simulink model "DCMotor_Lab4_Soln"  (R2023b)
settings: Solver=VariableStepAuto  StartTime=0.0  StopTime=5  MaxStep=0.001  RelTol=1e-3
PostLoadFcn:
  | % Resize the model window
  | set(0,"Units","pixels")
  | sSize = get(0,"screensize");
  | set_param(gcs,'location',...
  |     [1,sSize(4)*0.01,round(sSize(3)/2),sSize(4)*0.96]);
values from neighbouring files (symbols this model uses):
  m = 1000    [VehicleModelSoln.m]
  s = tf('s')    [PositionAnalysisSoln.m]
undefined symbols (not defined in the file or in its folder): X, Y, Z
libraries: sm_lib x22, fl_lib x10, nesl_utility x3, simulink_extras x1, simulink x1
settings Model: Creator=Rocksmithed  LastModifiedBy=callie
settings DebuggingCC: UnconnectedInputMsg=warning  UnconnectedOutputMsg=warning  UnconnectedLineMsg=warning
settings ModelReferenceCC: EnableRefExpFcnMdlSchedulingChecks=on
settings RTWCC: DLArmComputeVersion=19.05
settings ExplorerConfigSet: InternalSimMechanicsExplorerSettings="<ExplorerConfiguration><canonicalview>default</canonicalview><AnimationSetting><BasePlaybackSpeed>1.0</BasePlaybackSpeed><PlaybackSpeedFactor>1.0</PlaybackSpeedFactor></AnimationSetting><TilePanel><TileInfo><Tiles Columns=\"1\" Count=\"2\" Rows=\"2\"><Column Weight=\"1\"/><Row Weight=\"0.567\"/><Row Weight=\"0.433\"/><Tile Height=\"1\" Width=\"1\" X=\"0\" Y=\"0\"/><Tile Height=\"1\" Width=\"1\" X=\"0\" Y=\"1\"/></Tiles></TileInfo><SceneInfo><SceneViewer><BGColor><R>0.941176474094390869</R><G>0.941176474094390869</G><B>0.941176474094390869</B></BGColor><Camera><DoPerspective>off</DoPerspective><Position><X>-0.000930544299837629606</X><Y>-0.991947113333839781</Y><Z>-0.000895731694159566396</Z></Position><Center><X>-0.000930544299837629606</X><Y>0.00805288666616021942</Y><Z>-0.000895731694159566396</Z></Center><Up><X>0</X><Y>-0</Y><Z>1</Z></Up><ViewLimDist>1</ViewLimDist><YLim>0.032783521950277443</YLim><XLim>0.0566081835477763654</XLim></Camera></SceneViewer><SceneViewer><BGColor><R>0.941176474094390869</R><G>0.941176474094390869</G><B>0.941176474094390869</B></BGColor><Camera><DoPerspective>off</DoPerspective><Position><X>0.999997946466442578</X><Y>0.00754476683050594576</Y><Z>-0.00157074132845253563</Z></Position><Center><X>-2.05353355742232679e-06</X><Y>0.00754476683050594576</Y><Z>-0.00157074132845253563</Z></Center><Up><X>-0</X><Y>0</Y><Z>1</Z></Up><ViewLimDist>1</ViewLimDist><YLim>0.029549906028231071</YLim><XLim>0.0669823756881716137</XLim></Camera></SceneViewer></SceneInfo></TilePanel><MechEditorPanel><Cameras/><GfxPanelCameraMap/><VideoCreator><PlaybackSpeedRatio>1.0</PlaybackSpeedRatio><FrameRate>30</FrameRate><VideoFormat>Motion JPEG AVI</VideoFormat><FrameSize>auto</FrameSize></VideoCreator></MechEditorPanel></ExplorerConfiguration>"

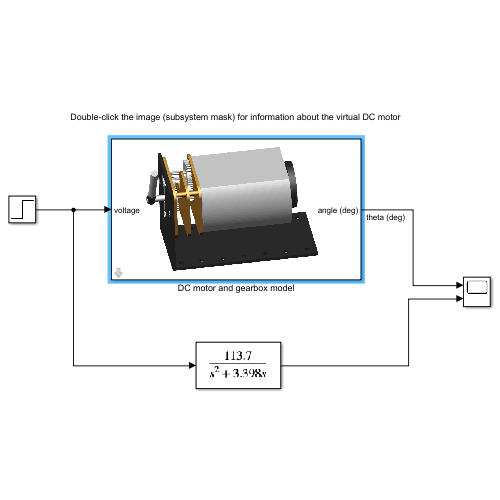
[thumbnail: Simulink's stored preview of the top-level diagram]
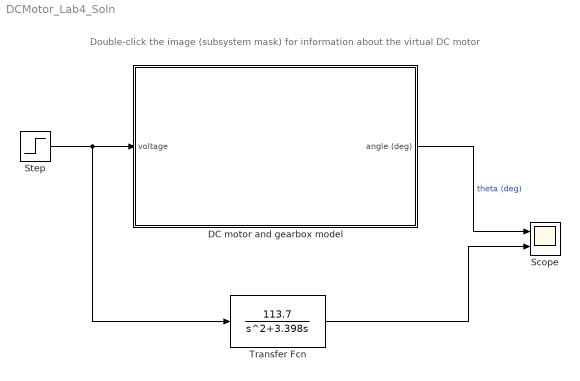
== system DCMotor_Lab4_Soln ==
  note: Double-click the image (subsystem mask) for information about the virtual DC motor
  DC motor and gearbox model : Subsystem  mask{B=0.028, K=0.05, L=0.1, R=0.25, noiseGain=0, saturationOn=off, pmass=0.150, plength=0.015}
      mask prompts: B "B: damping (N*m/(rad/s))"; K "K: constant of proportionality [V/(rad/s)]"; L "L: inductance (H)"; R "R: resistance (ohm)"; noiseGain "Sensor noise gain"; saturationOn "Use voltage saturation"; pmass "Pendulum mass (kg)"; plength "Pendulum length (m)"
      mask help:
      | This block implements a virtual DC motor using Simscape Multibody. The motor has a speed reducer with a 9:1 gear ratio.
      |
      | Inputs:
      |   voltage: the voltage applied to the motor in volts.
      | Outputs:
      |   angle: the angle of the output shaft in degrees.
      mask DialogControl Motor Prompt: Motor
      mask DialogControl Pendulum Prompt: Pendulum
      mask Display: image('dcmotor.png');
  Scope : Scope  NumInputPorts=2
  Step : Step  Time=0  SampleTime=0
  Transfer Fcn : TransferFcn  Numerator=[113.7]  Denominator=[1 3.398 0]
  wires:
  Step/1 -> Transfer Fcn/1, DC motor and gearbox model/1(voltage)
  DC motor and gearbox model/1(angle (deg)) -> Scope/1  "theta (deg)"
  Transfer Fcn/1 -> Scope/2

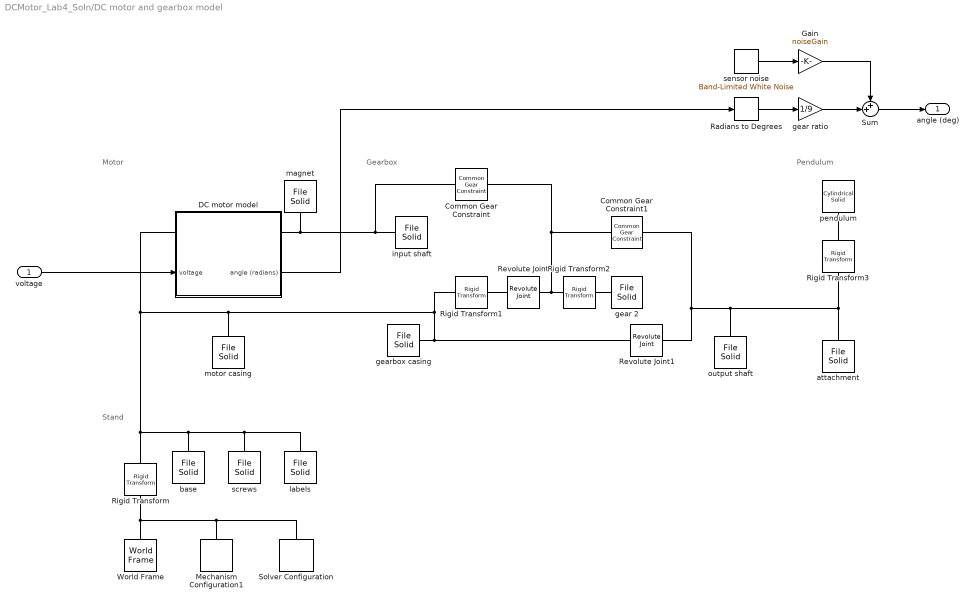
== system DCMotor_Lab4_Soln/DC motor and gearbox model ==
  note: Motor
  note: Stand
  note: Gearbox
  note: Pendulum
  voltage : Inport
  Common Gear Constraint : sm_lib/Gears and Couplings/Gears/Common Gear Constraint  GearType=External  SpecificationType=CenterDistanceRatio  CenterDistance=sqrt( 0.0046^2 + 0.0029^2 )  CenterDistanceUnits=m  GearRatio=3  BaseGearRadius=0.084  BaseGearRadiusUnits=m  FollGearRadius=0.084/3  FollGearRadiusUnits=cm  AssemblyGearRotation=Free
  Common Gear Constraint1 : sm_lib/Gears and Couplings/Gears/Common Gear Constraint  GearType=External  SpecificationType=CenterDistanceRatio  CenterDistance=sqrt( 0.0046^2 + 0.0029^2 )  CenterDistanceUnits=m  GearRatio=3  BaseGearRadius=0.084  BaseGearRadiusUnits=m  FollGearRadius=0.084/3  FollGearRadiusUnits=cm  AssemblyGearRotation=Free
  DC motor model : Subsystem
      settings: PortSchema="{\"entries\":[{\"content\":{\"sides\":[{\"content\":{\"connectorIds\":[\"LConn1\",\"In1\"]},\"type\":\"ConnectorPlacement.EquallySpacedRectSide\",\"uuid\":\"5a6d496b-9b68-4e77-90bc-41353dc42901\"},{\"content\":{\"connectorIds\":[\"RConn1\",\"Out1\"],\"side\":\"RIGHT\"},\"type\":\"ConnectorPlacement.EquallySpacedRectSide\",\"uuid\":\"9792b535-129a-41a8-a62b-92ba389600f0\"},{\"content\":{\"connectorIds\":[],\"side\":\"TOP\"},\"type\":\"ConnectorPlacement.EquallySpacedRectSide\",\"uuid\":\"2aab1536-3ac2-4e27-9370-d50050e6f4f6\"}]},\"type\":\"ConnectorPlacement.EquallySpacedConnector\",\"uuid\":\"df64eeb9-387f-493f-b882-741ae516d086\"}],\"packageUris\":[\"http://schema.mathworks.com/mf0/Connector/R2020b\"],\"version\":\"1.0\"}"
  Gain : Gain  Gain=noiseGain
  Mechanism Configuration1 : sm_lib/Utilities/Mechanism Configuration  UniformGravity=Constant  GravityVector=[0 0 -9.80665]  GravityVectorUnits=m/s^2  GravityUnits=m/s^2  LinearizationDelta=0.001  JointModeTransitionNonlinearIterations=2
  Radians to Degrees : simulink_extras/Transformations/Radians to Degrees
  Revolute Joint : sm_lib/Joints/Revolute Joint  JointMode=Normal  SenseConstraintForce=off  SenseConstraintForceX=off  SenseConstraintForceY=off  SenseConstraintForceZ=off  SenseConstraintTorque=off  SenseConstraintTorqueX=off  SenseConstraintTorqueY=off  SenseConstraintTorqueZ=off  SenseTotalForce=off  SenseTotalForceX=off  SenseTotalForceY=off  SenseTotalForceZ=off  SenseTotalTorque=off  SenseTotalTorqueX=off  SenseTotalTorqueY=off  SenseTotalTorqueZ=off  CompositeWrenchDir=FollowerOnBase  CompositeWrenchFrame=BaseFrame  EquilibriumPosition=0  EquilibriumPositionUnits=deg  SpringStiffness=0  SpringStiffnessUnits=N*m/deg  DampingCoefficient=0  DampingCoefficientUnits=N*m/(deg/s)  TorqueActuationMode=NoTorque  MotionActuationMode=ComputedMotion  SensePosition=off  SenseVelocity=off  SenseAcceleration=off  SenseTorqueForce=off  SenseLowerLimitTorqueForce=off  SenseUpperLimitTorqueForce=off  LowerLimitSpecify=off  LowerLimitBound=-90  LowerLimitBoundUnits=deg  LowerLimitStiffness=1e4  LowerLimitStiffnessUnits=N*m/deg  LowerLimitDamping=10  LowerLimitDampingUnits=N*m/(deg/s)  LowerLimitTransitionRegionWidth=0.1  LowerLimitTransitionRegionWidthUnits=deg  UpperLimitSpecify=off  UpperLimitBound=90  UpperLimitBoundUnits=deg  UpperLimitStiffness=1e4  UpperLimitStiffnessUnits=N*m/deg  UpperLimitDamping=10  UpperLimitDampingUnits=N*m/(deg/s)  UpperLimitTransitionRegionWidth=0.1  UpperLimitTransitionRegionWidthUnits=deg  PositionTargetSpecify=off  PositionTargetPriority=High  PositionTargetValue=0  PositionTargetValueUnits=deg  VelocityTargetSpecify=off  VelocityTargetPriority=High  VelocityTargetValue=0  VelocityTargetValueUnits=deg/s
  Revolute Joint1 : sm_lib/Joints/Revolute Joint  JointMode=Normal  SenseConstraintForce=off  SenseConstraintForceX=off  SenseConstraintForceY=off  SenseConstraintForceZ=off  SenseConstraintTorque=off  SenseConstraintTorqueX=off  SenseConstraintTorqueY=off  SenseConstraintTorqueZ=off  SenseTotalForce=off  SenseTotalForceX=off  SenseTotalForceY=off  SenseTotalForceZ=off  SenseTotalTorque=off  SenseTotalTorqueX=off  SenseTotalTorqueY=off  SenseTotalTorqueZ=off  CompositeWrenchDir=FollowerOnBase  CompositeWrenchFrame=BaseFrame  EquilibriumPosition=0  EquilibriumPositionUnits=deg  SpringStiffness=0  SpringStiffnessUnits=N*m/deg  DampingCoefficient=0  DampingCoefficientUnits=N*m/(deg/s)  TorqueActuationMode=NoTorque  MotionActuationMode=ComputedMotion  SensePosition=off  SenseVelocity=off  SenseAcceleration=off  SenseTorqueForce=off  SenseLowerLimitTorqueForce=off  SenseUpperLimitTorqueForce=off  LowerLimitSpecify=off  LowerLimitBound=-90  LowerLimitBoundUnits=deg  LowerLimitStiffness=1e4  LowerLimitStiffnessUnits=N*m/deg  LowerLimitDamping=10  LowerLimitDampingUnits=N*m/(deg/s)  LowerLimitTransitionRegionWidth=0.1  LowerLimitTransitionRegionWidthUnits=deg  UpperLimitSpecify=off  UpperLimitBound=90  UpperLimitBoundUnits=deg  UpperLimitStiffness=1e4  UpperLimitStiffnessUnits=N*m/deg  UpperLimitDamping=10  UpperLimitDampingUnits=N*m/(deg/s)  UpperLimitTransitionRegionWidth=0.1  UpperLimitTransitionRegionWidthUnits=deg  PositionTargetSpecify=off  PositionTargetPriority=High  PositionTargetValue=0  PositionTargetValueUnits=deg  VelocityTargetSpecify=off  VelocityTargetPriority=High  VelocityTargetValue=0  VelocityTargetValueUnits=deg/s
  Rigid Transform : sm_lib/Frames and Transforms/Rigid Transform  TranslationMethod=None  TranslationStandardOffset=0  TranslationLengthUnit=m  TranslationStandardAxis=+Z  TranslationCartesianOffset=[0 0 0]  TranslationROffset=0  TranslationROffsetUnits=m  TranslationZOffset=0  TranslationZOffsetUnits=m  TranslationThetaOffset=0  TranslationThetaOffsetUnits=deg  RotationMethod=StandardAxis  RotationAngleUnits=deg  RotationStandardAxis=+X  RotationAngle=90  RotationArbitraryAxis=[0 0 1]  FollAlignAxisA=+X  BaseAlignAxisA=+Y  FollAlignAxisB=+Y  BaseAlignAxisB=+Z  RotationSequenceAxes=FollowerAxes  RotationSequence=XYX  RotationSequenceAngles=[0 0 0]  RotationSequenceAnglesUnits=deg  RotationMatrix=[1 0 0; 0 1 0; 0 0 1]
  Rigid Transform1 : sm_lib/Frames and Transforms/Rigid Transform  TranslationMethod=Cartesian  TranslationStandardOffset=0  TranslationLengthUnit=m  TranslationStandardAxis=+Z  TranslationCartesianOffset=[-0.0046 0.0029 0]  TranslationROffset=0  TranslationROffsetUnits=m  TranslationZOffset=0  TranslationZOffsetUnits=m  TranslationThetaOffset=0  TranslationThetaOffsetUnits=deg  RotationMethod=None  RotationAngleUnits=deg  RotationStandardAxis=+Z  RotationAngle=0.0  RotationArbitraryAxis=[0 0 1]  FollAlignAxisA=+X  BaseAlignAxisA=+Y  FollAlignAxisB=+Y  BaseAlignAxisB=+Z  RotationSequenceAxes=FollowerAxes  RotationSequence=XYX  RotationSequenceAngles=[0 0 0]  RotationSequenceAnglesUnits=deg  RotationMatrix=[1 0 0; 0 1 0; 0 0 1]
  Rigid Transform2 : sm_lib/Frames and Transforms/Rigid Transform  TranslationMethod=Cartesian  TranslationStandardOffset=0  TranslationLengthUnit=m  TranslationStandardAxis=+Z  TranslationCartesianOffset=[-0.0046 0.0029 0]  TranslationROffset=0  TranslationROffsetUnits=m  TranslationZOffset=0  TranslationZOffsetUnits=m  TranslationThetaOffset=0  TranslationThetaOffsetUnits=deg  RotationMethod=None  RotationAngleUnits=deg  RotationStandardAxis=+Z  RotationAngle=0.0  RotationArbitraryAxis=[0 0 1]  FollAlignAxisA=+X  BaseAlignAxisA=+Y  FollAlignAxisB=+Y  BaseAlignAxisB=+Z  RotationSequenceAxes=FollowerAxes  RotationSequence=XYX  RotationSequenceAngles=[0 0 0]  RotationSequenceAnglesUnits=deg  RotationMatrix=[1 0 0; 0 1 0; 0 0 1]
  Rigid Transform3 : sm_lib/Frames and Transforms/Rigid Transform  TranslationMethod=Cartesian  TranslationStandardOffset=0  TranslationLengthUnit=m  TranslationStandardAxis=+Z  TranslationCartesianOffset=[0, -plength/2, 0.01075]  TranslationROffset=0  TranslationROffsetUnits=m  TranslationZOffset=0  TranslationZOffsetUnits=m  TranslationThetaOffset=0  TranslationThetaOffsetUnits=deg  RotationMethod=StandardAxis  RotationAngleUnits=deg  RotationStandardAxis=+X  RotationAngle=90  RotationArbitraryAxis=[0 0 1]  FollAlignAxisA=+X  BaseAlignAxisA=+Y  FollAlignAxisB=+Y  BaseAlignAxisB=+Z  RotationSequenceAxes=FollowerAxes  RotationSequence=XYX  RotationSequenceAngles=[0 0 0]  RotationSequenceAnglesUnits=deg  RotationMatrix=[1 0 0; 0 1 0; 0 0 1]
  Solver Configuration : nesl_utility/Solver Configuration  PhysicalDomain=network_engine_domain  SubClassName=solver  LeftPortType=input  RightPortType=generic  Tones=[]  Harmonics=[]  SimulateNoise=off  Profile=off  UseLocalSampling=off  EnableSwitchedLinearOptims=on  FrequencyDomain=off  UseCCode=off  RelTol=0.001  AbsTol=1e-06  MinStep=1e-09  ToWorkspace=off  RevertToSquareIcSolve=off  NumHomotopyIterations=100  PhasorMode=off  PhasorModeNumHarmonics=1  DoDC=off  ResidualTolerance=1e-09  UseLocalSolver=off  LocalSolverChoice=NE_BACKWARD_EULER_ADVANCER  LocalSolverSampleTime=0.001  DoFixedCost=off  MaxNonlinIter=3  MaxModeIter=2  ComputeImpulses=off  ImpulseIterations=2  LinearAlgebra=Sparse  EquationFormulation=NE_TIME_EF  DelaysMemoryBudget=1024  AutomaticFiltering=on  FilteringTimeConstant=0.001  PartitionStorageMethod=AS_NEEDED  PartitionMemoryBudget=1024  PartitionMethod=FAST
  Sum : Sum  Inputs=++|
  World Frame : sm_lib/Frames and Transforms/World Frame
  attachment : sm_lib/Body Elements/File Solid  ExtGeomFileName=dc_pendulumattachment.stl  UnitType=Custom  ExtGeomFileUnits=m  StepReaderType=HEX  ExportConvexHullGeometry=off  InertiaType=CalculateFromGeometry  Mass=1  MassUnits=kg  CenterOfMass=[0 0 0]  CenterOfMassUnits=m  MomentsOfInertia=[1 1 1]  MomentsOfInertiaUnits=kg*m^2  ProductsOfInertia=[0 0 0]  ProductsOfInertiaUnits=kg*m^2  BasedOnType=Density  Density=1000  DensityUnits=kg/m^3  DoExposeReferenceFrame=on  SerializedFrames=<Frames/>  GraphicType=FromGeometry  MarkerShape=Sphere  MarkerSize=10  GraphicVisPropType=AdvancedVisualProperties  GraphicDiffuseColor=[0.1 0.1 0.1 1]  GraphicSpecularColor=[0.9 0.9 0.9 1]  GraphicAmbientColor=[0.1 0.1 0.1 1]  GraphicEmissiveColor=[0 0 0 1]  GraphicShininess=10  GraphicOpacity=1.0
  base : sm_lib/Body Elements/File Solid  ExtGeomFileName=dc_stand.stl  UnitType=Custom  ExtGeomFileUnits=m  StepReaderType=HEX  ExportConvexHullGeometry=off  InertiaType=CalculateFromGeometry  Mass=1  MassUnits=kg  CenterOfMass=[0 0 0]  CenterOfMassUnits=m  MomentsOfInertia=[1 1 1]  MomentsOfInertiaUnits=kg*m^2  ProductsOfInertia=[0 0 0]  ProductsOfInertiaUnits=kg*m^2  BasedOnType=Density  Density=1000  DensityUnits=kg/m^3  DoExposeReferenceFrame=on  SerializedFrames=<Frames/>  GraphicType=FromGeometry  MarkerShape=Sphere  MarkerSize=10  GraphicVisPropType=AdvancedVisualProperties  GraphicDiffuseColor=[0.1 0.1 0.1 1]  GraphicSpecularColor=[0.9 0.9 0.9 1]  GraphicAmbientColor=[0.1 0.1 0.1 1]  GraphicEmissiveColor=[0 0 0 1]  GraphicShininess=10  GraphicOpacity=1.0
  gear 2 : sm_lib/Body Elements/File Solid  ExtGeomFileName=dc_gear2.stl  UnitType=Custom  ExtGeomFileUnits=m  StepReaderType=HEX  ExportConvexHullGeometry=off  InertiaType=CalculateFromGeometry  Mass=1  MassUnits=kg  CenterOfMass=[0 0 0]  CenterOfMassUnits=m  MomentsOfInertia=[1 1 1]  MomentsOfInertiaUnits=kg*m^2  ProductsOfInertia=[0 0 0]  ProductsOfInertiaUnits=kg*m^2  BasedOnType=Density  Density=1000  DensityUnits=kg/m^3  DoExposeReferenceFrame=on  SerializedFrames=<Frames/>  GraphicType=FromGeometry  MarkerShape=Sphere  MarkerSize=10  GraphicVisPropType=AdvancedVisualProperties  GraphicDiffuseColor=[1,1,1]  GraphicSpecularColor=[0.7 0.7 0.7]  GraphicAmbientColor=[0.2 0.2 0.2,1]  GraphicEmissiveColor=[0,0,0,1]  GraphicShininess=5  GraphicOpacity=1.0
  gear ratio : Gain  Gain=1/9
  gearbox casing : sm_lib/Body Elements/File Solid  ExtGeomFileName=dc_gearbox.stl  UnitType=Custom  ExtGeomFileUnits=m  StepReaderType=HEX  ExportConvexHullGeometry=off  InertiaType=CalculateFromGeometry  Mass=1  MassUnits=kg  CenterOfMass=[0 0 0]  CenterOfMassUnits=m  MomentsOfInertia=[1 1 1]  MomentsOfInertiaUnits=kg*m^2  ProductsOfInertia=[0 0 0]  ProductsOfInertiaUnits=kg*m^2  BasedOnType=Density  Density=1000  DensityUnits=kg/m^3  DoExposeReferenceFrame=on  SerializedFrames=<Frames/>  GraphicType=FromGeometry  MarkerShape=Sphere  MarkerSize=10  GraphicVisPropType=AdvancedVisualProperties  GraphicDiffuseColor=[1,0.85,0.2]  GraphicSpecularColor="[1    0.9   0.8 1]"  GraphicAmbientColor=[0.15 0.05 0.05 1]  GraphicEmissiveColor=[0.0 0.0 0.0 1.0]  GraphicShininess=5  GraphicOpacity=1.0
  input shaft : sm_lib/Body Elements/File Solid  ExtGeomFileName=dc_gear1.stl  UnitType=Custom  ExtGeomFileUnits=m  StepReaderType=HEX  ExportConvexHullGeometry=off  InertiaType=CalculateFromGeometry  Mass=1  MassUnits=kg  CenterOfMass=[0 0 0]  CenterOfMassUnits=m  MomentsOfInertia=[1 1 1]  MomentsOfInertiaUnits=kg*m^2  ProductsOfInertia=[0 0 0]  ProductsOfInertiaUnits=kg*m^2  BasedOnType=Density  Density=1000  DensityUnits=kg/m^3  DoExposeReferenceFrame=on  SerializedFrames=<Frames/>  GraphicType=FromGeometry  MarkerShape=Sphere  MarkerSize=10  GraphicVisPropType=AdvancedVisualProperties  GraphicDiffuseColor=[1,1,1]  GraphicSpecularColor=[0.7 0.7 0.7]  GraphicAmbientColor=[0.2 0.2 0.2,1]  GraphicEmissiveColor=[0,0,0,1]  GraphicShininess=5  GraphicOpacity=1.0
  labels : sm_lib/Body Elements/File Solid  ExtGeomFileName=dc_labels.stl  UnitType=Custom  ExtGeomFileUnits=m  StepReaderType=HEX  ExportConvexHullGeometry=off  InertiaType=CalculateFromGeometry  Mass=1  MassUnits=kg  CenterOfMass=[0 0 0]  CenterOfMassUnits=m  MomentsOfInertia=[1 1 1]  MomentsOfInertiaUnits=kg*m^2  ProductsOfInertia=[0 0 0]  ProductsOfInertiaUnits=kg*m^2  BasedOnType=Density  Density=1000  DensityUnits=kg/m^3  DoExposeReferenceFrame=on  SerializedFrames=<Frames/>  GraphicType=FromGeometry  MarkerShape=Sphere  MarkerSize=10  GraphicVisPropType=AdvancedVisualProperties  GraphicDiffuseColor=[0.95,0.95,0.95]  GraphicSpecularColor="[0.9    0.9  0.9 1]"  GraphicAmbientColor=[0.07 0.07 0.07]  GraphicEmissiveColor=[0.0 0.0 0.0 1.0]  GraphicShininess=2  GraphicOpacity=1.0
  magnet : sm_lib/Body Elements/File Solid  ExtGeomFileName=dc_magnet.stl  UnitType=Custom  ExtGeomFileUnits=m  StepReaderType=HEX  ExportConvexHullGeometry=off  InertiaType=CalculateFromGeometry  Mass=1  MassUnits=kg  CenterOfMass=[0 0 0]  CenterOfMassUnits=m  MomentsOfInertia=[1 1 1]  MomentsOfInertiaUnits=kg*m^2  ProductsOfInertia=[0 0 0]  ProductsOfInertiaUnits=kg*m^2  BasedOnType=Density  Density=1000  DensityUnits=kg/m^3  DoExposeReferenceFrame=on  SerializedFrames=<Frames/>  GraphicType=FromGeometry  MarkerShape=Sphere  MarkerSize=10  GraphicVisPropType=AdvancedVisualProperties  GraphicDiffuseColor=[0.1 0.1 0.1 1]  GraphicSpecularColor=[0.9 0.9 0.9 1]  GraphicAmbientColor=[0.1 0.1 0.1 1]  GraphicEmissiveColor=[0 0 0 1]  GraphicShininess=10  GraphicOpacity=1.0
  motor casing : sm_lib/Body Elements/File Solid  ExtGeomFileName=dc_motorcasing.stl  UnitType=Custom  ExtGeomFileUnits=m  StepReaderType=HEX  ExportConvexHullGeometry=off  InertiaType=CalculateFromGeometry  Mass=1  MassUnits=kg  CenterOfMass=[0 0 0]  CenterOfMassUnits=m  MomentsOfInertia=[1 1 1]  MomentsOfInertiaUnits=kg*m^2  ProductsOfInertia=[0 0 0]  ProductsOfInertiaUnits=kg*m^2  BasedOnType=Density  Density=1000  DensityUnits=kg/m^3  DoExposeReferenceFrame=on  SerializedFrames=<Frames/>  GraphicType=FromGeometry  MarkerShape=Sphere  MarkerSize=10  GraphicVisPropType=AdvancedVisualProperties  GraphicDiffuseColor=[1,1,1]  GraphicSpecularColor=[0.9 0.9 0.9]  GraphicAmbientColor=[0.3 0.3 0.3]  GraphicEmissiveColor=[0,0,0,1]  GraphicShininess=25  GraphicOpacity=1.0
  output shaft : sm_lib/Body Elements/File Solid  ExtGeomFileName=dc_outputshaft.stl  UnitType=Custom  ExtGeomFileUnits=m  StepReaderType=HEX  ExportConvexHullGeometry=off  InertiaType=CalculateFromGeometry  Mass=1  MassUnits=kg  CenterOfMass=[0 0 0]  CenterOfMassUnits=m  MomentsOfInertia=[1 1 1]  MomentsOfInertiaUnits=kg*m^2  ProductsOfInertia=[0 0 0]  ProductsOfInertiaUnits=kg*m^2  BasedOnType=Density  Density=1000  DensityUnits=kg/m^3  DoExposeReferenceFrame=on  SerializedFrames=<Frames/>  GraphicType=FromGeometry  MarkerShape=Sphere  MarkerSize=10  GraphicVisPropType=AdvancedVisualProperties  GraphicDiffuseColor=[1,1,1]  GraphicSpecularColor=[0.7 0.7 0.7]  GraphicAmbientColor=[0.2 0.2 0.2,1]  GraphicEmissiveColor=[0,0,0,1]  GraphicShininess=5  GraphicOpacity=1.0
  pendulum : sm_lib/Body Elements/Cylindrical Solid  GraphicAmbientColor=[0.3, 0.3, 0.3]  BasedOnType=Mass  CenterOfMass=[0 0 0]  CenterOfMassUnits=m  GraphicDiffuseColor=[1 1 1]  CylinderLength=plength  CylinderLengthUnits=m  CylinderRadius=0.0009  CylinderRadiusUnits=m  Density=1000  DensityUnits=kg/m^3  DoExposeReferenceFrame=on  GraphicEmissiveColor=[0.0 0.0 0.0 1.0]  ExportEntireGeometry=off  SerializedFrames=<Frames/>  MarkerShape=Sphere  MarkerSize=10  GraphicType=FromGeometry  InertiaType=CalculateFromGeometry  Mass=pmass  MassUnits=kg  MomentsOfInertia=[1 1 1]  MomentsOfInertiaUnits=kg*m^2  GraphicOpacity=1.0  ProductsOfInertia=[0 0 0]  ProductsOfInertiaUnits=kg*m^2  GraphicShininess=2  GraphicSpecularColor=[.1,0.1,0.1]  GraphicVisPropType=AdvancedVisualProperties
  screws : sm_lib/Body Elements/File Solid  ExtGeomFileName=dc_screws.stl  UnitType=Custom  ExtGeomFileUnits=m  StepReaderType=HEX  ExportConvexHullGeometry=off  InertiaType=CalculateFromGeometry  Mass=1  MassUnits=kg  CenterOfMass=[0 0 0]  CenterOfMassUnits=m  MomentsOfInertia=[1 1 1]  MomentsOfInertiaUnits=kg*m^2  ProductsOfInertia=[0 0 0]  ProductsOfInertiaUnits=kg*m^2  BasedOnType=Density  Density=1000  DensityUnits=kg/m^3  DoExposeReferenceFrame=on  SerializedFrames=<Frames/>  GraphicType=FromGeometry  MarkerShape=Sphere  MarkerSize=10  GraphicVisPropType=AdvancedVisualProperties  GraphicDiffuseColor=[0.95,0.95,0.95]  GraphicSpecularColor="[0.9    0.9  0.9 1]"  GraphicAmbientColor=[0.07 0.07 0.07]  GraphicEmissiveColor=[0.0 0.0 0.0 1.0]  GraphicShininess=2  GraphicOpacity=1.0
  sensor noise : simulink/Sources/Band-Limited White Noise  Cov=0.05  Ts=0.005  seed=[23341]
  angle (deg) : Outport
  wires:
  Gain/1 -> Sum/1
  Sum/1 -> angle (deg)/1
  gear ratio/1 -> Sum/2
  sensor noise/1 -> Gain/1
  Radians to Degrees/1 -> gear ratio/1
  DC motor model/1(angle (radians)) -> Radians to Degrees/1
  voltage/1 -> DC motor model/1(voltage)
  connections:
  attachment/RConn1 -- Rigid Transform3/LConn1 -- Common Gear Constraint1/RConn1 -- Revolute Joint1/RConn1 -- output shaft/RConn1
  Rigid Transform1/RConn1 -- Revolute Joint/LConn1
  Solver Configuration/RConn1 -- Mechanism Configuration1/RConn1 -- Rigid Transform/LConn1 -- World Frame/RConn1
  pendulum/RConn1 -- Rigid Transform3/RConn1
  DC motor model/RConn1 -- magnet/RConn1 -- Common Gear Constraint/LConn1 -- input shaft/RConn1
  Revolute Joint/RConn1 -- Common Gear Constraint1/LConn1 -- Common Gear Constraint/RConn1 -- Rigid Transform2/RConn1
  gear 2/RConn1 -- Rigid Transform2/LConn1
  DC motor model/LConn1 -- gearbox casing/RConn1 -- Revolute Joint1/LConn1 -- Rigid Transform1/LConn1 -- motor casing/RConn1 -- Rigid Transform/RConn1 -- screws/RConn1 -- labels/RConn1 -- base/RConn1

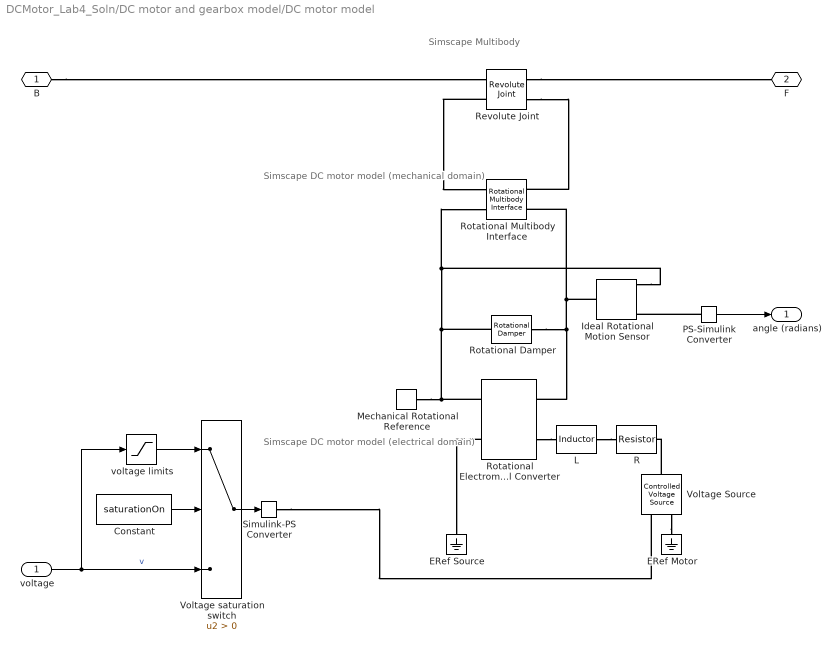
== system DCMotor_Lab4_Soln/DC motor and gearbox model/DC motor model ==
  note: Simscape Multibody
  note: Simscape DC motor model
      | (mechanical domain)
  note: Simscape DC motor model
      | (electrical domain)
  voltage : Inport
  Constant : Constant  Value=saturationOn
  ERef Motor : fl_lib/Electrical/Electrical Elements/Electrical Reference
  ERef Source : fl_lib/Electrical/Electrical Elements/Electrical Reference
  Ideal Rotational Motion Sensor : fl_lib/Mechanical/Mechanical Sensors/Ideal Rotational Motion Sensor  wrap_angle=simscape.enum.onoff.off  offset=0 rad
  L : fl_lib/Electrical/Electrical Elements/Inductor  l=L H  r=0 Ohm  g=1e-09 1/Ohm  i_specify=off  i_priority=High  i=0 A  i_nominal_specify=off  i_nominal_unit=A  i_nominal_value=1  v_specify=off  v_priority=High  v=0 V  v_nominal_specify=off  v_nominal_unit=V  v_nominal_value=1  i_L_specify=on  i_L_priority=High  i_L=0 A  i_L_nominal_specify=off  i_L_nominal_unit=A  i_L_nominal_value=1
  Mechanical Rotational Reference : fl_lib/Mechanical/Rotational Elements/Mechanical Rotational Reference
  PS-Simulink Converter : nesl_utility/PS-Simulink Converter  PhysicalDomain=network_engine_domain  SubClassName=ps_output  LeftPortType=input  RightPortType=output  PseudoPeriodic=off  Frequencies=[]  Unit=inherit  AffineConversion=off
  R : fl_lib/Electrical/Electrical Elements/Resistor  Tag=Factory Generic  R=R Ohm  i_specify=off  i_priority=High  i=0 A  i_nominal_specify=off  i_nominal_unit=A  i_nominal_value=1  v_specify=off  v_priority=High  v=0 V  v_nominal_specify=off  v_nominal_unit=V  v_nominal_value=1
  Revolute Joint : sm_lib/Joints/Revolute Joint  JointMode=Normal  SenseConstraintForce=off  SenseConstraintForceX=off  SenseConstraintForceY=off  SenseConstraintForceZ=off  SenseConstraintTorque=off  SenseConstraintTorqueX=off  SenseConstraintTorqueY=off  SenseConstraintTorqueZ=off  SenseTotalForce=off  SenseTotalForceX=off  SenseTotalForceY=off  SenseTotalForceZ=off  SenseTotalTorque=off  SenseTotalTorqueX=off  SenseTotalTorqueY=off  SenseTotalTorqueZ=off  CompositeWrenchDir=FollowerOnBase  CompositeWrenchFrame=BaseFrame  EquilibriumPosition=0  EquilibriumPositionUnits=deg  SpringStiffness=0  SpringStiffnessUnits=N*m/deg  DampingCoefficient=0  DampingCoefficientUnits=N*m/(deg/s)  TorqueActuationMode=InputTorque  MotionActuationMode=ComputedMotion  SensePosition=off  SenseVelocity=on  SenseAcceleration=off  SenseTorqueForce=off  SenseLowerLimitTorqueForce=off  SenseUpperLimitTorqueForce=off  LowerLimitSpecify=off  LowerLimitBound=-90  LowerLimitBoundUnits=deg  LowerLimitStiffness=1e4  LowerLimitStiffnessUnits=N*m/deg  LowerLimitDamping=10  LowerLimitDampingUnits=N*m/(deg/s)  LowerLimitTransitionRegionWidth=0.1  LowerLimitTransitionRegionWidthUnits=deg  UpperLimitSpecify=off  UpperLimitBound=90  UpperLimitBoundUnits=deg  UpperLimitStiffness=1e4  UpperLimitStiffnessUnits=N*m/deg  UpperLimitDamping=10  UpperLimitDampingUnits=N*m/(deg/s)  UpperLimitTransitionRegionWidth=0.1  UpperLimitTransitionRegionWidthUnits=deg  PositionTargetSpecify=off  PositionTargetPriority=High  PositionTargetValue=90  PositionTargetValueUnits=deg  VelocityTargetSpecify=off  VelocityTargetPriority=High  VelocityTargetValue=0  VelocityTargetValueUnits=deg/s
  Rotational Electromechanical Converter : fl_lib/Electrical/Electrical Elements/Rotational Electromechanical Converter  K=K V/(rad/s)  i_specify=off  i_priority=High  i=0 A  i_nominal_specify=off  i_nominal_unit=A  i_nominal_value=1  v_specify=off  v_priority=High  v=0 V  v_nominal_specify=off  v_nominal_unit=V  v_nominal_value=1  t_specify=off  t_priority=High  t=0 N*m  t_nominal_specify=off  t_nominal_unit=N*m  t_nominal_value=1  w_specify=off  w_priority=High  w=0 rad/s  w_nominal_specify=off  w_nominal_unit=rad/s  w_nominal_value=1
  Rotational Damper : fl_lib/Mechanical/Rotational Elements/Rotational Damper  D=B N*m/(rad/s)  w_specify=off  w_priority=None  w=0 rad/s  w_nominal_specify=off  w_nominal_unit=rad/s  w_nominal_value=1  t_specify=off  t_priority=None  t=0 N*m  t_nominal_specify=off  t_nominal_unit=N*m  t_nominal_value=1
  Rotational Multibody Interface : fl_lib/Mechanical/Multibody Interfaces/Rotational Multibody Interface
  Simulink-PS Converter : nesl_utility/Simulink-PS Converter  PhysicalDomain=network_engine_domain  SubClassName=ps_input  LeftPortType=input  RightPortType=output  PseudoPeriodic=off  Frequencies=[]  NoiseDistribution=none  NoiseParameters=[]  Unit=1  AffineConversion=off  FilteringAndDerivatives=zero  SimscapeFilterOrder=1  InputFilterTimeConstant=0.005  UdotUserProvided=1
  Voltage Source : fl_lib/Electrical/Electrical Sources/Controlled Voltage Source
  Voltage saturation switch : Switch  Criteria=u2 > Threshold  SaturateOnIntegerOverflow=off  InputSameDT=off
  voltage limits : Saturate  UpperLimit=24  LowerLimit=-24
  B : PMIOPort  Side=Left
  F : PMIOPort  Port=2  Side=Right
  angle (radians) : Outport
  wires:
  Constant/1 -> Voltage saturation switch/2
  voltage limits/1 -> Voltage saturation switch/1
  PS-Simulink Converter/1 -> angle (radians)/1
  Voltage saturation switch/1 -> Simulink-PS Converter/1
  voltage/1 -> voltage limits/1, Voltage saturation switch/3  "v"
  connections:
  Voltage Source/LConn1 -- R/LConn1
  Voltage Source/RConn2 -- ERef Motor/LConn1
  Revolute Joint/LConn2 -- Rotational Multibody Interface/LConn1
  Revolute Joint/RConn2 -- Rotational Multibody Interface/RConn1
  Revolute Joint/RConn1 -- F/RConn1
  B/RConn1 -- Revolute Joint/LConn1
  PS-Simulink Converter/LConn1 -- Ideal Rotational Motion Sensor/RConn3
  Rotational Electromechanical Converter/LConn2 -- Rotational Multibody Interface/RConn2 -- Ideal Rotational Motion Sensor/LConn1 -- Rotational Damper/LConn1
  Rotational Damper/RConn1 -- Rotational Multibody Interface/LConn2 -- Ideal Rotational Motion Sensor/RConn1 -- Rotational Electromechanical Converter/RConn2 -- Mechanical Rotational Reference/LConn1
  Simulink-PS Converter/RConn1 -- Voltage Source/RConn1
  L/LConn1 -- R/RConn1
  Rotational Electromechanical Converter/LConn1 -- L/RConn1
  Rotational Electromechanical Converter/RConn1 -- ERef Source/LConn1
